simulink model "PassVeh14DOF"  (R2026b)
settings: Solver=ode23tb  StopTime=inf  FixedStep=.001  RelTol=1e-1  EnableMultiTasking=on
model workspace (MAT data in the model file):
  AlgnTrqCambCompl = [0 0 0 0]
  AlgnTrqSteerCompl = [0 0 0 0]
  AxlIxx = 62.3745166667
  AxlM = 160
  BumpCamber = [0 0 0 0]
  BumpCaster = [0 0 0 0]
  BumpSteer = [0 0 0 0]
  CambVsSteerAng = [0 0 0 0]
  CastVsSteerAng = [0 0 0 0]
  Cps = 2
  Cz = 5565.2246438
  CzWhlAxl = 11490.971257
  DCT_Param.Transmission.Ratios = [3.78 2.18 1.43 1.03 0.935 0.84]
  DCT_Param.Transmission.Shaft_Inertia_Odd = 0.0023
  DCT_Param.Transmission.Shaft_Inertia_Even = 0.0009
  DCT_Param.Transmission.Shaft_Inertia_Output = 0.008
  DCT_Param.Transmission.Gear_Inertia = 0.001
  DCT_Param.Transmission.Gear_Efficiency = 0.94
  DCT_Param.Transmission.Gear_Ang_Vel_Thr = 0.01
  DCT_Param.Transmission.Shaft_Velocity_Odd = 0
  DCT_Param.Transmission.Shaft_Velocity_Even = 0
  DCT_Param.Transmission.Shaft_Velocity_Output = 0
  DCT_Param.Transmission.Gear_Initial_Velocity = 0
  DCT_Param.Transmission.Abstract.Compliance = 100000
  DCT_Param.Transmission.Abstract.Damping = 10000
  DCT_Param.Transmission.Abstract.Ratio_Time_Const = 0.05
  DCT_Param.Transmission.Abstract.Shift_Gear_Delay = 25
  DCT_Param.Clutch.Torque_Radius = 130
  DCT_Param.Clutch.Num_Friction_Surfaces = 4
  DCT_Param.Clutch.Engagement_Piston_Area = 0.001
  DCT_Param.Clutch.Kinetic_Friction_Coeff = 0.3
  DCT_Param.Clutch.Static_Friction_Coeff = 0.31
  DCT_Param.Clutch.Derating_Factor = 1
  DCT_Param.Clutch.Clutch_Velocity_Tolerance = 0.001
  DCT_Param.Clutch.Threshold_Pressure = 1
  DCT_Param.Clutch.Drag_Torque_Coeff = 0
  DCT_Param.Dog_Clutch.Max_Torque = 1000
  DCT_Param.Dog_Clutch.Teeth_Mean_Radius = 50
  DCT_Param.Dog_Clutch.Tooth_Height = 10
  DCT_Param.Dog_Clutch.Ring_Hub_Clearance = 3
  DCT_Param.Dog_Clutch.Ring_Stop_Stiffness = 1000000
  DCT_Param.Dog_Clutch.Ring_Stop_Damping = 1000
  DCT_Param.Dog_Clutch.Shift_Linkage_Damping = 100
  DCT_Param.Dog_Clutch.Max_Engage_Velocity = 1000000
  DCT_Param.Dog_Clutch.Tooth_Engage_Overlap = 3
  DCT_Param.Vehicle.Mass = 1600
  DCT_Param.Vehicle.Wheels_Per_Axle = 2
  DCT_Param.Vehicle.Distance_CG_FrontAxle = 1.7
  DCT_Param.Vehicle.Distance_CG_RearAxle = 2
  DCT_Param.Vehicle.Distance_CG_Ground = 0.5
  DCT_Param.Vehicle.Frontal_Area = 3
  DCT_Param.Vehicle.Aero_Drag_Coeff = 0.4
  DCT_Param.Vehicle.Initial_Velocity = 0
  DCT_Param.Vehicle.Final_Drive_Ratio = 3.7
  DCT_Param.Vehicle.Final_Drive_Efficiency = 0.86
  DCT_Param.Vehicle.Final_Drive_Vel_Thresh = 0.01
  DCT_Param.Vehicle.Side_Shaft_Inertia = 0.01
  DCT_Param.Vehicle.Side_Shaft_Initial_Velocity = 0
  DCT_Param.Vehicle.Tire.Radius = 0.312
  DCT_Param.Vehicle.Tire.Inertia = 0.5
  DCT_Param.Vehicle.Tire.Initial_Velocity = 0
  DCT_Param.Vehicle.Tire.Slip_Vel_Thresh = 0.1
  DCT_Param.Vehicle.Tire.Nominal_Vertical_Load = 4000
  DCT_Param.Vehicle.Tire.C_Coeff = 1.685
  DCT_Param.Vehicle.Tire.D_Coeff = [1.21 -0.037]
  DCT_Param.Vehicle.Tire.E_Coeff = [0.344 0.095 -0.02 0]
  DCT_Param.Vehicle.Tire.BCD_Coeff = [21.51 -0.163 0.245]
  DCT_Param.Vehicle.Tire.H_Coeff = [-0.002 0.002]
  DCT_Param.Vehicle.Tire.V_Coeff = [0 0]
  DCT_Param.ICE.Max_Power = 100000
  DCT_Param.ICE.Speed_At_Max_Power = 5500
  DCT_Param.ICE.Max_Speed = 7000
  DCT_Param.ICE.Stall_Speed = 200
  DCT_Param.ICE.Shaft_Inertia = 0.2
  DCT_Param.ICE.Initial_Velocity = 800
  DCT_Param.ICE.Idle_Ref_Spd = 800
  DCT_Param.ICE.Engine_Time_Constant = 0.2
  DCT_Param.ICE.Initial_Normalized_Throttle = 0
  DCT_Param.ICE.Speed_Threshold = 20
  DCT_Param.ICE.FC.Speed_Vector = [0 368.421052632 736.842105263 1105.26315789 1473.68421053 1842.10526316 2210.52631579 2578.94736842 2947.36842105 3315.78947368 3684.21052632 4052.63157895 4421.05263158 4789.47368421 5157.89473684 5526.31578947 5894.73684211 6263.15789474 6631.57894737 7000]
  DCT_Param.ICE.FC.Torque_Vector = [0 10.5263157895 21.0526315789 31.5789473684 42.1052631579 52.6315789474 63.1578947368 73.6842105263 84.2105263158 94.7368421053 105.263157895 115.789473684 126.315789474 136.842105263 147.368421053 157.894736842 168.421052632 178.947368421 189.473684211 200]
  DCT_Param.ICE.FC.Consumption_Table = [0.262945178015 0.225304787522 0.201465019624 0.191425874321 0.195187351614 0.212749451502 0.244112173984 0.289275519063 0.348239486736 0.421004077004 0.507569289868 0.607935125326 ... (400 elements, 20x20)]
  DCT_Param.Shift_Map_Example.Pedal_Positions = [0.1 0.4 0.5 0.9]
  DCT_Param.Shift_Map_Example.Upshift_Speeds = [11  20  26  34.5  43; 14  26  35  44.5  55; 17  31  42  52.5  65; 21  39  52  66.5  80]
  DCT_Param.Shift_Map_Example.Downshift_Speeds = [8.9  17  23.6  32.4  40.8; 11.5  22.7  32  41.6  52.2; 14  27  38.1  50  62; 18  33  48  62.6  76.2]
  DCT_Param.Shift_Map_ORIG.Pedal_Positions = [0.1 0.4 0.5 0.9]
  DCT_Param.Shift_Map_ORIG.Upshift_Speeds = [11.5  23.5  35.5  45.5  55.5; 14.5  26.5  38.5  48.5  58.5; 17.5  29.5  41.5  51.5  61.5; 20.5  32.5  44.5  54.5  64.5]
  DCT_Param.Shift_Map_ORIG.Downshift_Speeds = [8.5  20.5  32.5  42.5  52.5; 11.5  23.5  35.5  45.5  55.5; 14.5  26.5  38.5  48.5  58.5; 17.5  29.5  41.5  51.5  61.5]
  DCT_Param.Shift_Map_OPT.Pedal_Positions = [0.1 0.4 0.5 0.9]
  DCT_Param.Shift_Map_OPT.Upshift_Speeds = [17.8469  29.8469  35.8159  41.2981  46.3004; 19.2469  33.9778  43.9778  53.9778  63.9778; 24.5469  41.9778  62.1778  78.5778  106.9778; 27.5469  59.3778  99.0445  109.0445  119.0445]
  DCT_Param.Shift_Map_OPT.Downshift_Speeds = [14.8469  26.8469  32.8159  38.2981  43.3004; 16.2469  30.9778  40.9778  50.9778  60.9778; 21.5469  38.9778  59.1778  75.5778  103.9778; 24.5469  56.3778  96.0445  106.0445  116.0445]
  DCT_Param.Shift_Map.Pedal_Positions = [0.1 0.4 0.5 0.9]
  DCT_Param.Shift_Map.Upshift_Speeds = [11.5  23.5  35.5  45.5  55.5; 14.5  26.5  38.5  48.5  58.5; 17.5  29.5  41.5  51.5  61.5; 20.5  32.5  44.5  54.5  64.5]
  DCT_Param.Shift_Map.Downshift_Speeds = [8.5  20.5  32.5  42.5  52.5; 11.5  23.5  35.5  45.5  55.5; 14.5  26.5  38.5  48.5  58.5; 17.5  29.5  41.5  51.5  61.5]
  DCT_Param.Control.Clutch.Min_Lock_Pressure = 2000000
  DCT_Param.Control.Clutch.Max_Lock_Pressure = 5000000
  DCT_Param.Control.Clutch.Max_Unlock_Pressure = 500000
  DCT_Param.Control.Engine_Start_RPM = 800
  DCT_Param.Control.Engine_Stop_RPM = 790
  DCT_Param.Control.Mode_Logic_TS = 0.1
  DCT_Param.Control.ICE.Kp = 0.02
  DCT_Param.Control.ICE.Ki = 0.01
  DCT_Param.Control.Gen.Kp = 10
  DCT_Param.Control.Gen.Ki = 3
  DCT_Param.Control.Mot.Kp = 500
  DCT_Param.Control.Mot.Ki = 300
  DCT_Param.Control.Veh_Spd.Kp = 0.02
  DCT_Param.Control.Veh_Spd.Ki = 0.04
  DCT_Param.Driver.Kp = 400
  DCT_Param.Driver.Ki = 0.001
  DCT_Param.Driver.Pedal_Filter_Const = 0.01
  DCT_Param.Dog_Clutches.Pulse_Delay = 50
  DCT_Param.Dog_Clutches.Pulse_Length = 20
  DCT_Param.Animation.Teeth_Ratios = [0.338461538462 0.555555555556 0.916666666667 0.96 1.17948717949 1.92307692308]
  DCT_Param.Animation.Teeth_Ratios_Reverse = [0.458333333333 0.75]
  DCT_Param.Shift_Map_OPT506.Pedal_Positions = [0.1 0.4 0.5 0.9]
  DCT_Param.Shift_Map_OPT506.Upshift_Speeds = [18  30.2  48.3  67.3322  77.3429; 20.1  36.85  66.6178  76.7537  86.7537; 21.1  40.25  71.0189  81.0189  91.7873; 24.1  63.75  80.7523  105.9489  115.9489]
  DCT_Param.Shift_Map_OPT506.Downshift_Speeds = [15  27.2  45.3  64.3322  74.3429; 17.1  33.85  63.6178  73.7537  83.7537; 18.1  37.25  68.0189  78.0189  88.7873; 21.1  60.75  77.7523  102.9489  112.9489]
  DCT_Param.Shift_Map_OPTAbsRea176.Pedal_Positions = [0.1 0.4 0.5 0.9]
  DCT_Param.Shift_Map_OPTAbsRea176.Upshift_Speeds = [17.8469  29.8469  35.7875  44.0901  49.4243; 18.9219  34.1312  45.8256  59.7585  69.7585; 32.1719  43.4585  53.51  103.2151  114.6401; 35.1719  59.2585  99.5217  109.5217  119.5217]
  DCT_Param.Shift_Map_OPTAbsRea176.Downshift_Speeds = [14.8469  26.8469  32.7875  41.0901  46.4243; 15.9219  31.1312  42.8256  56.7585  66.7585; 29.1719  40.4585  50.51  100.2151  111.6401; 32.1719  56.2585  96.5217  106.5217  116.5217]
  Downshift_Speeds = [9.5625  23.0625  36.5625  47.8125  59.0625  68.90625  78.75; 12.9375  26.4375  39.9375  51.1875  62.4375  72.84375  83.25; 16.3125  29.8125  43.3125  54.5625  65.8125  76.78125  87.75; 19.6875  33.1875  46.6875  57.9375  69.1875  80.71875  92.25]
  F0z = [2886 2907]
  F0zWhlAxl = 2907
  Hmax = 0.25
  Kz = 52451.0065793
  KzWhlAxl = 138031.612078
  LatCambCompl = [0 0 0 0]
  LatSteerCompl = [0 0 0 0]
  LatWhlCtrComplLat = [0 0 0 0]
  LatWhlCtrComplLng = [0  0  0  0; 0  0  0  0]
  LatWhlCtrDisp = [0 0 0 0]
  LngCambCompl = [0  0  0  0; 0  0  0  0]
  LngCastCompl = [0  0  0  0; 0  0  0  0]
  LngSteerCompl = [0  0  0  0; 0  0  0  0]
  LngWhlCtrCompl = [0  0  0  0; 0  0  0  0]
  LngWhlCtrDisp = [0 0 0 0]
  MotRatios = [1 1]
  NCyl = 6
  NrmlWhlFrcOff = [2886 2886 2907 2907]
  NrmlWhlRates = [52.4510065793 52.4510065793 52.4510065793 52.4510065793]
  Pedal_Positions = [0.1 0.4 0.5 0.9]
  Pstd = 101325
  Rair = 287
  RollCamber.RL = [-10  -1; 0  0; 10  1]
  RollCamber.RR = [-10  1; 0  0; 10  -1]
  RollCaster.RL = [-10  -1; 0  0; 10  1]
  RollCaster.RR = [-10  1; 0  0; 10  -1]
  RollSteer.RL = [-10  -1; 0  0; 10  1]
  RollSteer.RR = [-10  1; 0  0; 10  -1]
  RollStiffArb = [0 0]
  RollStiffArbFrnt = 800
  RollStiffNoArb = [0 0]
  RollStiffNoArbFrnt = 0
  RollStiffNoTwstRear = 0
  ShckFrcVsCompRate = [5.5652246438 5.5652246438 5.5652246438 5.5652246438]
  StatCamber = [0 0 0 0]
  StatCaster = [0 0 0 0]
  StatLdWhlR = [0.3 0.3 0.3 0.3]
  StatToe = [0 0 0 0]
  Trans.InputShaftInertia = 0.01
  Trans.InputShaftDamping = 0.001
  Trans.FinalDrive = 2.77
  Trans.GearRatios = [-3.82 4.56 4.56 2.97 2.08 1.69 1.27 1 0.85 0.65]
  Trans.GearNums = [-1 0 1 2 3 4 5 6 7 8]
  Trans.Inertias = [0.128 0.01 0.128 0.1 0.062 0.028 0.01 0.01 0.01 0.01]
  Trans.DampingCoeffs = [0.003 0.001 0.003 0.0025 0.002 0.001 0.001 0.001 0.001 0.001]
  Trans.Efficiencies = [0.9 0.9 0.9 0.9 0.9 0.95 0.95 0.95 0.95 0.95]
  Trans.ShiftTau = 0.01
  Tstd = 293.15
  Upshift_Speeds = [12.9375  26.4375  39.9375  51.1875  62.4375  72.84375  83.25; 16.3125  29.8125  43.3125  54.5625  65.8125  76.78125  87.75; 19.6875  33.1875  46.6875  57.9375  69.1875  80.71875  92.25; 33  52.5  77.25  100.5  138.75  161.875  185]
  VEH.Mass = 1181
  VEH.StaticNormalFrontLoad.FR = 264.666666667
  VEH.StaticNormalFrontLoad.FL = 264.666666667
  VEH.StaticNormalRearLoad.RR = 322
  VEH.StaticNormalRearLoad.RL = 322
  VEH.WheelBase = 3.075
  VEH.FrontAxlePositionfromCG = 1.515
  VEH.RearAxlePositionfromCG = 1.504
  VEH.HeightCG = 0.134
  VEH.FrontalArea = 2.11
  VEH.DragCoefficient = 0.33
  VEH.NumberOfWheelsPerAxle = 2
  VEH.PitchMomentInertia = 1922.66666667
  VEH.RollMomentInertia = 432.333333333
  VEH.YawMomentInertia = 2066
  VEH.SteeringRatio = 18
  VEH.TrackWidth = 1.922
  VEH.SprungMass = 1096.72266667
  VEH.InitialLongPosition = 0
  VEH.InitialLatPosition = 0
  VEH.InitialVertPosition = 0
  VEH.InitialRollAngle = 0
  VEH.InitialPitchAngle = 0
  VEH.InitialYawAngle = 0
  VEH.InitialLongVel = 0
  VEH.InitialLatVel = 0
  VEH.InitialVertVel = 0
  VEH.InitialRollRate = 0
  VEH.InitialPitchRate = 0
  VEH.InitialYawRate = 0
  VEH.UnsprungMassRearAxle = 160
  VEH.UnsprungMassFrontAxle = 100
  Vd = 0.00346
  VrtLdTrnsfr = [0 0 0 0]
  WH.Mass = 11.4333333333
  dt3D = 0.05
  f_air = [0 0 0 0 0 0 0 0 0 0 0 0 ... (256 elements, 16x16)]
  f_co = [0 0 0 0 0 0 0 0 0 0 0 0 ... (256 elements, 16x16)]
  f_co2 = [0 0 0 0 0 0 0 0 0 0 0 0 ... (256 elements, 16x16)]
  f_eff = [352.135682859 352.135682859 320.724378192 303.655312657 295.930136708 291.240087194 291.240271258 291.240312459 291.240275452 291.240198499 291.240100781 291.240018769 ... (256 elements, 16x16)]
  f_fuel = [0 0 0 0 0 0 0 0 0 0 0 0 ... (256 elements, 16x16)]
  f_hc = [0 0 0 0 0 0 0 0 0 0 0 0 ... (256 elements, 16x16)]
  f_nox = [0 0 0 0 0 0 0 0 0 0 0 0 ... (256 elements, 16x16)]
  f_pm = [0  0  0  0  0  0  0  0  0  0  0  0  0  0  0  0; 0  0  0  0  0  0  0  0  0  0  0  0  0  0  0  0; 0  0  0  0  0  0  0  0  0  0  0  0  0  0  0  0; 0  0  0  0  0  0  0  0  0  0  0  0  0  0  0  0; 0  0  0  0  0  0  0  0  0  0  0  0  0  0  0  0; 0  0  0  0  0  0  0  0  0  0  0  0  0  0  0  0; 0  0  0  0  0  0  0  0  0  0  0  0  0  0  0  0; 0  0  0  0  0  0  0  0  0  0  0  0  0  0  0  0; 0  0  0  0  0  0  0  0  0  0  0  0  0  0  0  0; 0  0  0  0  0  0  0  0  0  0  0  0  0  0  0  0; 0  0  0  0  0  0  0  0  0  0  0  0  0  0  0  0; 0  0  0  0  0  0  0  0  0  0  0  0  0  0  0  0; 0  0  0  0  0  0  0  0  0  0  0  0  0  0  0  0; 0  0  0  0  0  0  0  0  0  0  0  0  0  0  0  0; 0  0  0  0  0  0  0  0  0  0  0  0  0  0  0  0; 0  0  0  0  0  0  0  0  0  0  0  0  0  0  0  0]
  f_susp_axl_bp = [1 2]
  f_susp_dz_bp = [-0.325022776267 -0.315022776267 -0.305022776267 -0.205022776267 -0.105022776267 -0.00502277626717 0.0949772237328 0.194977223733 0.204977223733 0.214977223733]
  f_susp_dzdot_bp = [-3 -0.3 -0.2 -0.1 0 0.1 0.2 0.3 3]
  f_susp_fmz = [-144070.391448 -93629.24037 -75929.1118915 -20630.5828179 -15385.48216 -10140.3815021 -4895.28084414 349.819813785 -31916.3973792 18437.6709544 -83996.1993354 -33555.0482577 ... (43920 elements, 10x9x61x2x4)]
  f_susp_geom = [0 0 0 0 0 0 0 0 0 0 0 0 ... (3660 elements, 10x61x2x3)]
  f_susp_strgdelta_bp = [-0.523598775598 -0.506145483078 -0.488692190558 -0.471238898038 -0.453785605519 -0.436332312999 -0.418879020479 -0.401425727959 -0.383972435439 -0.366519142919 -0.349065850399 -0.331612557879 -0.314159265359 -0.296705972839 -0.279252680319 -0.261799387799 -0.244346095279 -0.226892802759 -0.209439510239 -0.191986217719 -0.174532925199 -0.157079632679 -0.13962634016 -0.12217304764 -0.10471975512 -0.0872664625997 -0.0698131700798 -0.0523598775598 -0.0349065850399 -0.0174532925199 0 0.0174532925199 0.0349065850399 0.0523598775598 0.0698131700798 0.0872664625997 0.10471975512 0.12217304764 0.13962634016 0.157079632679 0.174532925199 0.191986217719 0.209439510239 0.226892802759 0.244346095279 0.261799387799 0.279252680319 0.296705972839 0.314159265359 0.331612557879 0.349065850399 0.366519142919 0.383972435439 0.401425727959 0.418879020479 0.436332312999 0.453785605519 0.471238898038 0.488692190558 0.506145483078 0.523598775598]
  f_tbrake = [0 76.8593923996 105.140482948 131.533638111 157.926793274 176.658631717 176.65727296 176.656856686 176.656879077 176.657093756 176.657404516 176.65772406 ... (256 elements, 16x16)]
  f_tbrake_n_bpt = [0 649.519052838 912.419621844 1175.32019085 1438.22075986 1701.12132886 1964.02189787 2226.92246687 2489.82303588 2752.72360489 3015.62417389 3278.5247429 3541.4253119 3804.32588091 4067.22644992 4330.12701892]
  f_tbrake_t_bpt = [0 34.6410161514 61.0341713143 87.4273264773 113.82048164 140.213636803 166.606791966 192.999947129 219.393102292 245.786257455 272.179412618 298.572567781 324.965722944 351.358878107 377.75203327 404.145188433]
  f_texh = [766.752464599 766.752464599 786.17542386 801.679939032 884.591982581 910.574397722 910.571871054 910.570774534 910.570601632 910.570821151 910.571247242 910.571639815 ... (256 elements, 16x16)]
  f_twc_eff_co = [0.17 0.25 0.45 0.99 0.99 0.99 0.99]
  f_twc_eff_hc = [0.21 0.375 0.75 0.98 0.98 0.98 0.98]
  f_twc_eff_lam = [0.909090909 0.944055944 0.979020979 1 1.013986014 1.048951049 1.083916084]
  f_twc_eff_nox = [0.98 0.98 0.98 0.97 0.05 0.02 0]
  numWheel = 4
libraries: vehdynlibtire x12, vehdynlibsuspension x8, autolibutils x5, sharedtransform x5, shared6dof x2, vehdynlibeom x1, vehdynlibtirecommon x1, matrix_library x1
(part 1 of 9)
settings Model: DataDictionary=PassVeh14DOF.sldd  ModifiedByFormat=The MathWorks, Inc.  SimulationMode=accelerator  Creator=The MathWorks, Inc.  LastModifiedBy=The MathWorks, Inc.
settings SolverCC: DecoupledContinuousIntegration=on  SolverJacobianMethodControl=FullPerturbation  ZeroCrossAlgorithm=Adaptive
settings DataIOCC: ReturnWorkspaceOutputs=off
settings OptimizationCC: ReuseModelBlockBuffer=off
settings DebuggingCC: ArithmeticOperatorsInVariantConditions=warning  ArtificialAlgebraicLoopMsg=none  IgnoredZcDiagnostic=none  MaskedZcDiagnostic=none  PregeneratedLibrarySubsystemCodeDiagnostic=none  SubsystemReferenceDiagnosticForUnitTest=warning
settings ModelReferenceCC: ModelReferenceMinAlgLoopOccurrences=on
settings SFSimCC: CustomCodeUndefinedFunction=UseInterfaceOnly  SimUseLocalCustomCode=off
settings RTWCC: DLArmComputeVersion=19.05  LargeConstantGeneration=WriteOnlyDNNConstantsToDataFiles  RTWUseLocalCustomCode=off

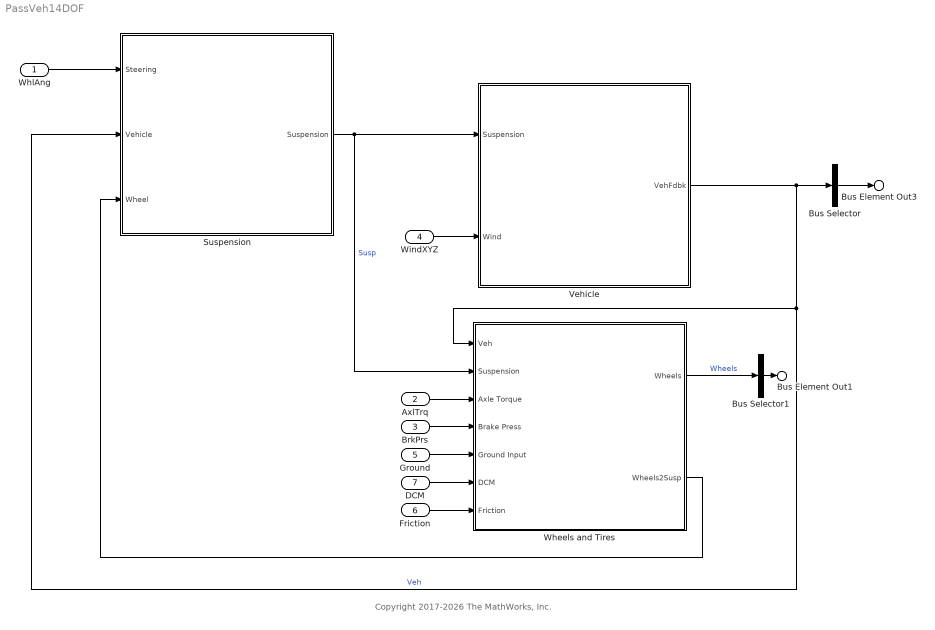
== system PassVeh14DOF ==
  note: Copyright 2017-2026 The MathWorks, Inc.
  WhlAng : Inport  Unit=rad  PortDimensions=4
  AxlTrq : Inport  Port=2  Unit=N*m  PortDimensions=4
  BrkPrs : Inport  Port=3  PortDimensions=4
  WindXYZ : Inport  Port=4  Unit=m/s  PortDimensions=3
  Ground : Inport  Port=5  Unit=m  PortDimensions=4
  Friction : Inport  Port=6  Unit=1  PortDimensions=4
  DCM : Inport  Port=7  PortDimensions=[3,3,4]
  Bus Selector : BusSelector  OutputSignals=InertFrm,BdyFrm  OutputAsBus=on
  Bus Selector1 : BusSelector  OutputSignals=TireFrame,Steering  OutputAsBus=on
  Suspension : Subsystem  Variant=on  VariantControlMode=label  LabelModeActiveChoice=3
      mask Display:
      | switch str2num(get_param(gcb,'ActiveVariant'))
      |     case 1
      |         image('suspdw.png');
      |     case 2
      |         image([imread('suspindmap.png');imread('suspsamap.png')]);
      |     case 3
      |          image([imread('suspmacp.png');imread('suspsacoil.png')]);
      |     case 4
      |          image('suspmacp.png');
      |     case 5
      |          image('suspindmap.png');
      |     case 6
      |          image('suspkandc.png');
      | end
  Vehicle : Subsystem
      mask Display: image('6dofcar.png');
  Wheels and Tires : Subsystem
      mask Display: image('wheel3dof.png')
  Bus Element Out3 : Outport  PortName=Veh
  Bus Element Out1 : Outport  Port=2  PortName=Wheels
  wires:
  Vehicle/1(VehFdbk) -> Bus Selector/1, Wheels and Tires/1(Veh), Suspension/2(Vehicle)  "Veh"
  WhlAng/1 -> Suspension/1(Steering)
  WindXYZ/1 -> Vehicle/2(Wind)
  Suspension/1(Suspension) -> Vehicle/1(Suspension), Wheels and Tires/2(Suspension)  "Susp"
  Wheels and Tires/1(Wheels) -> Bus Selector1/1  "Wheels"
  Ground/1 -> Wheels and Tires/5(Ground Input)
  BrkPrs/1 -> Wheels and Tires/4(Brake Press)
  AxlTrq/1 -> Wheels and Tires/3(Axle Torque)
  Friction/1 -> Wheels and Tires/7(Friction)
  Bus Selector/1 -> Bus Element Out3/1
  Bus Selector1/1 -> Bus Element Out1/1
  Wheels and Tires/2(Wheels2Susp) -> Suspension/3(Wheel)
  DCM/1 -> Wheels and Tires/6(DCM)
